simulink model "FOC_core"  (R2025b)
settings: Solver=FixedStepAuto  StartTime=0.0  StopTime=Tstop  FixedStep=p.FastTs  RelTol=1e-3
undefined symbols (not defined in the file): angleDeg, c, Inverter, Motor, p, torqueNm
libraries: fl_lib x4, nesl_utility x3, simulink x2, ee_lib x1
Description:
  | Release 3.0.2
settings Model: Creator=dehc5899  LastModifiedBy=dehc5899
settings SolverCC: AutoInsertRateTranBlk=on
settings DebuggingCC: UnderspecifiedInitializationDetection=Classic

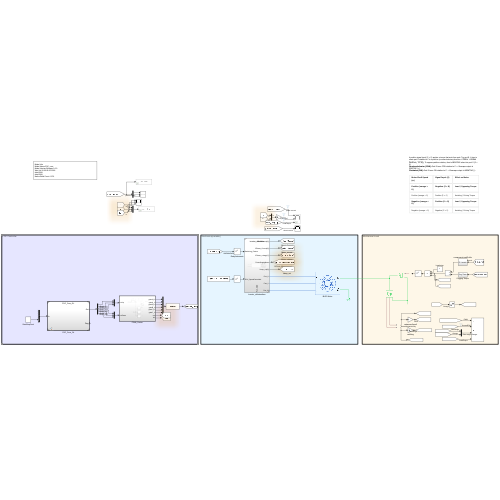
[thumbnail: Simulink's stored preview of the top-level diagram]
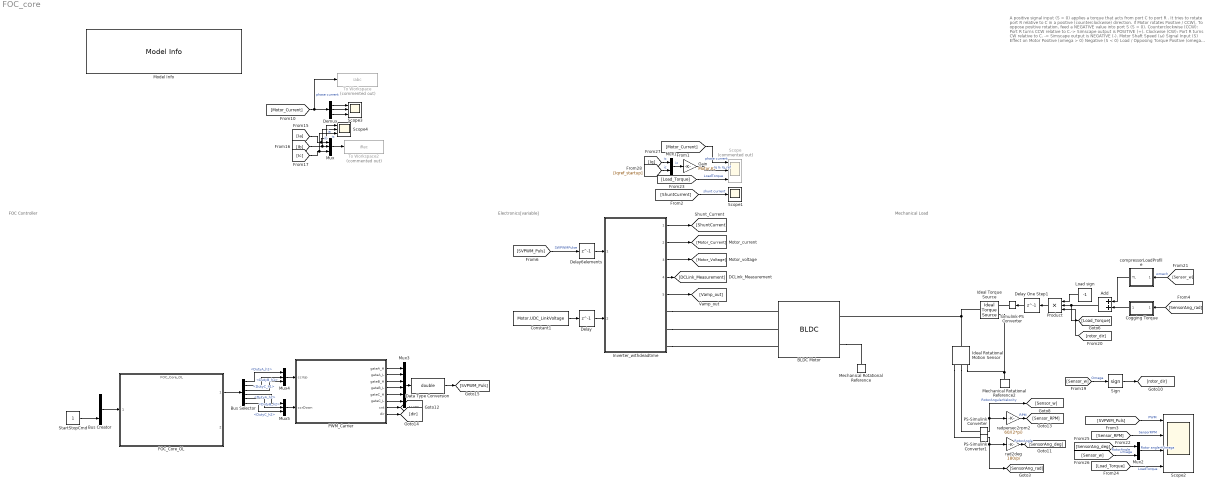
== system FOC_core ==
  note: FOC Controller
  note: A positive signal input (S > 0) applies a torque that acts from port C to port R . It tries to rotate port R relative to C in a positive (counterclockwise) direction. if Motor rotates Positive / CCW), To oppose positive rotation, feed a NEGATIVE value into port S (S < 0).
      | Counterclockwise (CCW): Port R turns CCW relative to C.-> Simscape output is POSITIVE (+).
      | Clockwise (CW): Port R turns CW relative to C. -> Simscape output is NEGATIVE (-).
      |
      | Motor Shaft Speed (ω)
      | Signal Input (S)
      | Effect on Motor
      |
      | Positive (omega > 0)
      | Negative (S < 0)
      | Load / Opposing Torque
      |
      | Positive (omega > 0)
      | Positive (S > 0)
      | Assisting / Driving Torque
      |
      | Negative (omega < 0)
      | Positive (S > 0)
      | Load / Opposing Torque
      |
      | Negative (omega < 0)
      | Negative (S < 0)
      | Assisting / Driving Torque
  note: Electronics[variable]
  note: Mechanical Load
  Add : Sum
  BLDC Motor : ee_lib/Electromechanical/Permanent Magnet/BLDC  port_option=ee.enum.threePhasePort.expanded  rotor_param=ee.enum.pmsm.backemf.tabulatedbackemf  pm_flux_linkage=0.03 Wb  theta_constant=pi / 12 rad  emf_max=9.6 V  w_meas=Motor.bemfMeasSpeed rpm  DphiDtheta_tab=[0, -.1528, -.1528, .1528, .1528, 0] Wb/rad  back_emf_tab=BEMF_shape V  rotor_angle_tab=theta_mech deg  nPolePairs=Motor.PP_NumberOfPolePairs  axes_param=ee.enum.rotorangle.daxis  winding_type=ee.enum.electromech.statorconfiguration.wye  stator_param=ee.enum.statorparam.LsLmMs  machine_param=ee.enum.dqparameterization.constant  Ld=0.00022 H  Lq=0.00022 H  idVec=[-200, 0, 200] A  iqVec=[-200, 0, 200] A  LdMatrix=0.00022 * ones(3, 3) H  LqMatrix=0.00022 * ones(3, 3) H  L0=0.00016 H  Ls=Motor.Ls H  Lm=Motor.Lm H  Ms=Motor.Ms H  Rs=Motor.R_StatorResistance Ohm  zero_sequence=ee.enum.park.zerosequence.exclude  loss_param=ee.enum.ironloss.empirical  losses_oc=[0, 0, 0] W  losses_sc=[0, 0, 0] W  f_losses=60 Hz  Isc_losses=95 A  J=Motor.J_Inertia kg*m^2  lam=Motor.F_FrictionCoeff N*m*s/rad  i_d_specify=off  i_d_priority=None  i_d=0 A  i_d_nominal_specify=off  i_d_nominal_value=1  i_d_nominal_unit=A  i_q_specify=off  i_q_priority=None  i_q=0 A  i_q_nominal_specify=off  i_q_nominal_value=1  i_q_nominal_unit=A  torque_specify=off  torque_priority=None  torque=0 N*m  torque_nominal_specify=off  torque_nominal_value=1  torque_nominal_unit=N*m  angular_velocity_specify=on  angular_velocity_priority=Low  angular_velocity=Motor.wm0_InitialRotorSpeed rpm  angular_velocity_nominal_specify=off  angular_velocity_nominal_value=Motor.nNom_NominalSpeedrpm  angular_velocity_nominal_unit=rpm  angular_position_specify=on  angular_position_priority=Low  angular_position=Motor.thm0_InitialRotorAngle rad  angular_position_nominal_specify=off  angular_position_nominal_value=Motor.thm0_InitialRotorAngle  angular_position_nominal_unit=deg  alpha=3.93e-3 1/K  alpha_flux=-0.001 1/K  Tmeas=298.15 K  stator_thermal_mass=100 J/K  rotor_thermal_mass=200 J/K  Rm_percent_rotor=90  Rd_percent_rotor=30  temperatureA_specify=off  temperatureA_priority=High  temperatureA=25 degC  temperatureA_nominal_specify=off  temperatureA_nominal_value=1  temperatureA_nominal_unit=degC  temperatureB_specify=off  temperatureB_priority=High  temperatureB=25 degC  temperatureB_nominal_specify=off  temperatureB_nominal_value=1  temperatureB_nominal_unit=degC  temperatureC_specify=off  temperatureC_priority=High  temperatureC=25 degC  temperatureC_nominal_specify=off  temperatureC_nominal_value=1  temperatureC_nominal_unit=degC  temperatureR_specify=off  temperatureR_priority=High  temperatureR=25 degC  temperatureR_nominal_specify=off  temperatureR_nominal_value=1  temperatureR_nominal_unit=degC
      settings: InternalSimscapePortConfiguration="{\"Bottom\":[],\"Left\":[{\"id\":\"a\",\"label\":\"a\",\"type\":\"foundation.electrical.electrical\"},{\"id\":\"b\",\"label\":\"b\",\"type\":\"foundation.electrical.electrical\"},{\"id\":\"c\",\"label\":\"c\",\"type\":\"foundation.electrical.electrical\"}],\"Right\":[{\"id\":\"R\",\"label\":\"R\",\"type\":\"foundation.mechanical.rotational.rotational\"},{\"id\":\"C\",\"label\":\"C\",\"type\":\"foundation.mechanical.rotational.rotational\"}],\"Top\":[]}"
  Bus Creator : BusCreator  Inputs=7  OutDataTypeStr=Bus: FOC_Inputs_t
  Bus Selector : BusSelector  OutputSignals=DutyA_h1,DutyB_h1,DutyC_h1,DutyA_h2,DutyB_h2,DutyC_h2
  Cogging Torque : Subsystem
      settings: PortSchema="{\"entries\":[{\"content\":{\"sides\":[{\"content\":{\"connectorIds\":[\"Out1\"]},\"type\":\"ConnectorPlacement.EquallySpacedRectSide\",\"uuid\":\"e72dd149-be6c-473d-b9a6-ab382dc36dd8\"},{\"content\":{\"connectorIds\":[\"In1\"],\"side\":\"RIGHT\"},\"type\":\"ConnectorPlacement.EquallySpacedRectSide\",\"uuid\":\"d6dbddf8-c929-46f7-8e18-d8605da261d8\"},{\"content\":{\"side\":\"TOP\"},\"type\":\"ConnectorPlacement.EquallySpacedRectSide\",\"uuid\":\"d97b9a66-7b14-44a9-8763-71570facd52d\"},{\"content\":{\"side\":\"BOTTOM\"},\"type\":\"ConnectorPlacement.EquallySpacedRectSide\",\"uuid\":\"30e90f76-fd4e-40c6-9e4e-ba219d693512\"}]},\"type\":\"ConnectorPlacement.EquallySpacedConnector\",\"uuid\":\"ce9d67e2-aed0-4e64-a6bd-15c2f7731a50\"}],\"packageUris\":[\"http://schema.mathworks.com/mf0/Connector/R2020b\"],\"version\":\"1.0\"}"
  Constant1 : Constant  Value=Motor.UDC_LinkVoltage
  Data Type Conversion : DataTypeConversion  OutDataTypeStr=double  SaturateOnIntegerOverflow=off  RndMeth=Floor
  Delay : Delay  DelayLength=1  InitialCondition=Inverter.UDC_LinkVoltage_Max  InputProcessing=Columns as channels (frame based)
  Delay One Step1 : Delay  DelayLength=1
  Delay6elements : Delay  DelayLength=1  InitialCondition=[0 0 0 0 0 0]
  Demux : Demux  Outputs=3
  FOC_Core_OL : ModelReference  ModelNameDialog=FOC_Core_OL  SimulationMode=Normal  ModelReferenceVersion=1.291
  Gain : Gain  Gain=Motor.Kt
  Ideal Rotational Motion Sensor : fl_lib/Mechanical/Mechanical Sensors/Ideal Rotational Motion Sensor  reference=foundation.enum.MeasurementReference.difference  acceleration_port=false  velocity_port=true  position_port=true  wrap_angle=true  offset=Motor.thm0_InitialRotorAngle rad
  Ideal Torque Source : fl_lib/Mechanical/Mechanical Sources/Ideal Torque Source
  Inverter_withdeadtime : Subsystem  ReferencedSubsystem=inverter_withdtime
      settings: PortSchema="{\"entries\":[{\"content\":{\"sides\":[{\"content\":{\"connectorIds\":[\"In1\",\"In2\"]},\"type\":\"ConnectorPlacement.EquallySpacedRectSide\",\"uuid\":\"c4e4a499-a73b-47b6-b9d4-05a0b5c00da1\"},{\"content\":{\"connectorIds\":[\"Out1\",\"Out2\",\"Out3\",\"Out4\",\"Out5\",\"RConn1\",\"RConn2\",\"RConn3\"],\"side\":\"RIGHT\"},\"type\":\"ConnectorPlacement.EquallySpacedRectSide\",\"uuid\":\"f55443ed-1206-46a2-9a95-70ed1e950cf9\"},{\"content\":{\"side\":\"TOP\"},\"type\":\"ConnectorPlacement.EquallySpacedRectSide\",\"uuid\":\"cf76199e-050b-45cf-ab73-853bf2c84fa8\"},{\"content\":{\"connectorIds\":[\"RConn4\"],\"side\":\"BOTTOM\"},\"type\":\"ConnectorPlacement.EquallySpacedRectSide\",\"uuid\":\"91869a37-cdc1-4525-aadb-c80a51613b54\"}]},\"type\":\"ConnectorPlacement.EquallySpacedConnector\",\"uuid\":\"fb7c01bd-e96a-47ac-9a1b-b2a6f4f5bd80\"}],\"packageUris\":[\"http://schema.mathworks.com/mf0/Connector/R2020b\"],\"version\":\"1.0\"}"
  Load sign : Constant  Value=-1
  Mechanical Rotational Reference : fl_lib/Mechanical/Rotational Elements/Mechanical Rotational Reference
  Mechanical Rotational Reference2 : fl_lib/Mechanical/Rotational Elements/Mechanical Rotational Reference
  Model Info : simulink/Model-Wide Utilities/Model Info  Frame=on  DisplayStringWithTags=|  HorizontalTextAlignment=Left  LeftAlignmentValue=0.02
      | Model Info
      | Model Name:%<ModelName>
      | Model Version:%<Description>
      | %<Created>
      | %<Creator>
      | %<LastModifiedBy>
      | Native Build Count:%<ModelVersion>
  Mux : Mux  Inputs=3
  Mux1 : Mux  Inputs=2
  Mux2 : Mux  Inputs=2
  Mux3 : Mux  Inputs=6
  Mux4 : Mux  Inputs=3
  Mux5 : Mux  Inputs=3
  PS-Simulink Converter : nesl_utility/PS-Simulink Converter  PhysicalDomain=network_engine_domain  SubClassName=ps_output  LeftPortType=input  RightPortType=output  PseudoPeriodic=off  Frequencies=[]  VectorFormat=inherit  Unit=inherit  AffineConversion=off
  PS-Simulink Converter1 : nesl_utility/PS-Simulink Converter  PhysicalDomain=network_engine_domain  SubClassName=ps_output  LeftPortType=input  RightPortType=output  PseudoPeriodic=off  Frequencies=[]  VectorFormat=inherit  Unit=inherit  AffineConversion=off
  PWM_Carrier : Subsystem  TreatAsAtomicUnit=on  SystemSampleTime=p.FastTs
  Product : Product  Inputs=3
  Scope : Scope  Commented=on  NumInputPorts=3
      settings: ActiveDisplayYMinimum=-25.470769165207408  ActiveDisplayYMaximum=27.204092861454868  DataLoggingVariableName=ScopeData4
  Scope1 : Scope
      settings: ActiveDisplayYMinimum=-6.3618713706725121  ActiveDisplayYMaximum=11.690256831370988  DataLoggingVariableName=ScopeData9
  Scope2 : Scope  NumInputPorts=4
      settings: ActiveDisplayYMinimum=-0.12499999999999997  ActiveDisplayYMaximum=1.125  DataLoggingVariableName=ScopeData5
  Scope3 : Scope  NumInputPorts=3
      settings: ActiveDisplayYMinimum=-12.058935324686422  ActiveDisplayYMaximum=12.950717402584473  DataLoggingVariableName=ScopeData23
  Scope4 : Scope  NumInputPorts=3
      settings: ActiveDisplayYMinimum=-2.083290326404279  ActiveDisplayYMaximum=1.1649120394540577  DataLoggingVariableName=ScopeData17
  Sign : Signum
  Simulink-PS Converter : nesl_utility/Simulink-PS Converter  PhysicalDomain=network_engine_domain  SubClassName=ps_input  LeftPortType=input  RightPortType=output  PseudoPeriodic=off  Frequencies=[]  NoiseDistribution=none  NoiseParameters=[]  Unit=1  AffineConversion=off  FilteringAndDerivatives=provide  SimscapeFilterOrder=1  InputFilterTimeConstant=0.001  UdotUserProvided=0
  StartStopCmd : Constant  OutDataTypeStr=uint8
  To Workspace : ToWorkspace  Commented=on  VariableName=iabc  SaveFormat=Timeseries  SampleTime=-1
  To Workspace2 : ToWorkspace  Commented=on  VariableName=iRec  SaveFormat=Timeseries  SampleTime=-1
  compressorLoadProfile : Subsystem
  rad2deg : Gain  Gain=180/pi
  radpersec2rpm2 : Gain  Gain=60/(2*pi)
  wires:
  Inverter_withdeadtime/4 -> [DCLink_Measurement]
  [SVPWM_Puls] -> Delay6elements/1  "SWPWMPulse"
  Inverter_withdeadtime/3 -> [Motor_Voltage]
  Inverter_withdeadtime/2 -> [Motor_Current]
  Inverter_withdeadtime/1 -> [ShuntCurrent]
  Delay/1 -> Inverter_withdeadtime/2
  Constant1/1 -> Delay/1
  Delay6elements/1 -> Inverter_withdeadtime/1
  [SensorAng_rad] -> Cogging Torque/1(Theta)
  PS-Simulink Converter/1 -> radpersec2rpm2/1, [Sensor_w]  "RotorAngularVelocity"
  rad2deg/1 -> [SensorAng_deg]  "RotorAngle"
  [Load_Torque] -> Scope2/4  "LoadTorque"
  PS-Simulink Converter1/1 -> [SensorAng_rad], rad2deg/1
  [Sensor_w] -> Mux2/2  "Omega"
  Cogging Torque/1(Tcog) -> Add/2
  Add/1 -> Product/2, [Load_Torque]
  [SensorAng_deg] -> Mux2/1  "RotorAngle"
  [SVPWM_Puls] -> Scope2/1  "PWM"
  radpersec2rpm2/1 -> [Sensor_RPM]  "RPM"
  Mux2/1 -> Scope2/3  "Rotor angle+Omega"
  [Sensor_RPM] -> Scope2/2  "SensorRPM"
  [Motor_Current] -> Scope/1  "phase current"
  [ShuntCurrent] -> Scope1/1  "shunt current"
  Inverter_withdeadtime/5 -> [Vamp_out]
  [Ib] -> Scope4/2, Mux/2  "ib"
  [Ia] -> Scope4/1, Mux/1  "ia"
  [Ic] -> Scope4/3, Mux/3  "ic"
  [Motor_Current] -> To Workspace/1, Demux/1  "phase current"
  Demux/1 -> Scope3/1
  Demux/2 -> Scope3/2
  Demux/3 -> Scope3/3
  Mux/1 -> To Workspace2/1
  Product/1 -> Delay One Step1/1
  [Sensor_w] -> Sign/1  "Omega"
  Sign/1 -> [rotor_dir]
  Load sign/1 -> Product/1
  [rotor_dir] -> Product/3
  Delay One Step1/1 -> Simulink-PS Converter/1
  [Sensor_w] -> compressorLoadProfile/1(wmech)  "wmech"
  compressorLoadProfile/1(TL) -> Add/1
  [Load_Torque] -> Scope/3  "LoadTorque"
  Mux1/1 -> Gain/1  "ic"
  Gain/1 -> Scope/2  "Iq & Iq_ref"
  [Iq] -> Mux1/1  "ic"
  [Iqref_startup] -> Mux1/2  "ic"
  PWM_Carrier/2(gateA_L) -> Mux3/2
  PWM_Carrier/5(gateC_H) -> Mux3/5
  PWM_Carrier/1(gateA_H) -> Mux3/1
  PWM_Carrier/7(cnt) -> [cnt]
  PWM_Carrier/6(gateC_L) -> Mux3/6
  PWM_Carrier/3(gateB_H) -> Mux3/3
  PWM_Carrier/4(gateB_L) -> Mux3/4
  Data Type Conversion/1 -> [SVPWM_Puls]
  PWM_Carrier/8(dir) -> [dir]
  Mux3/1 -> Data Type Conversion/1
  FOC_Core_OL/1 -> Bus Selector/1
  Bus Creator/1 -> FOC_Core_OL/1
  Mux4/1 -> PWM_Carrier/1(ccrUp)
  Bus Selector/1 -> Mux4/1  "<DutyA_h1>"
  Bus Selector/2 -> Mux4/2  "<DutyB_h1>"
  Bus Selector/3 -> Mux4/3  "<DutyC_h1>"
  Bus Selector/4 -> Mux5/1  "<DutyA_h2>"
  Bus Selector/5 -> Mux5/2  "<DutyB_h2>"
  Bus Selector/6 -> Mux5/3  "<DutyC_h2>"
  Mux5/1 -> PWM_Carrier/2(ccrDown)
  StartStopCmd/1 -> Bus Creator/6
  connections:
  BLDC Motor/RConn2 -- Mechanical Rotational Reference/LConn1
  Inverter_withdeadtime/RConn1 -- BLDC Motor/LConn1
  Inverter_withdeadtime/RConn2 -- BLDC Motor/LConn2
  Inverter_withdeadtime/RConn3 -- BLDC Motor/LConn3
  Mechanical Rotational Reference2/LConn1 -- Ideal Rotational Motion Sensor/RConn1 -- Ideal Torque Source/RConn2
  Ideal Torque Source/LConn1 -- Ideal Rotational Motion Sensor/LConn1 -- BLDC Motor/RConn1
  Ideal Rotational Motion Sensor/RConn3 -- PS-Simulink Converter1/LConn1
  Ideal Rotational Motion Sensor/RConn2 -- PS-Simulink Converter/LConn1
  Simulink-PS Converter/RConn1 -- Ideal Torque Source/RConn1

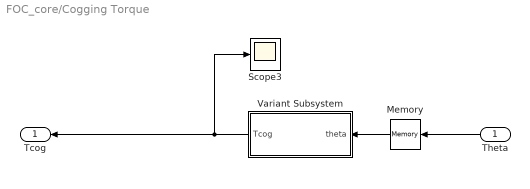
== system FOC_core/Cogging Torque ==
  Theta : Inport
  Memory : Memory
  Scope3 : Scope
      settings: ActiveDisplayYMinimum=-0.048749999766971877  ActiveDisplayYMaximum=0.048749999963062271  DataLoggingVariableName=ScopeData6
  Variant Subsystem : Subsystem  Variant=on  EmptyChoice=on
  Tcog : Outport
  wires:
  Theta/1 -> Memory/1
  Variant Subsystem/1(Tcog) -> Scope3/1, Tcog/1
  Memory/1 -> Variant Subsystem/1(theta)

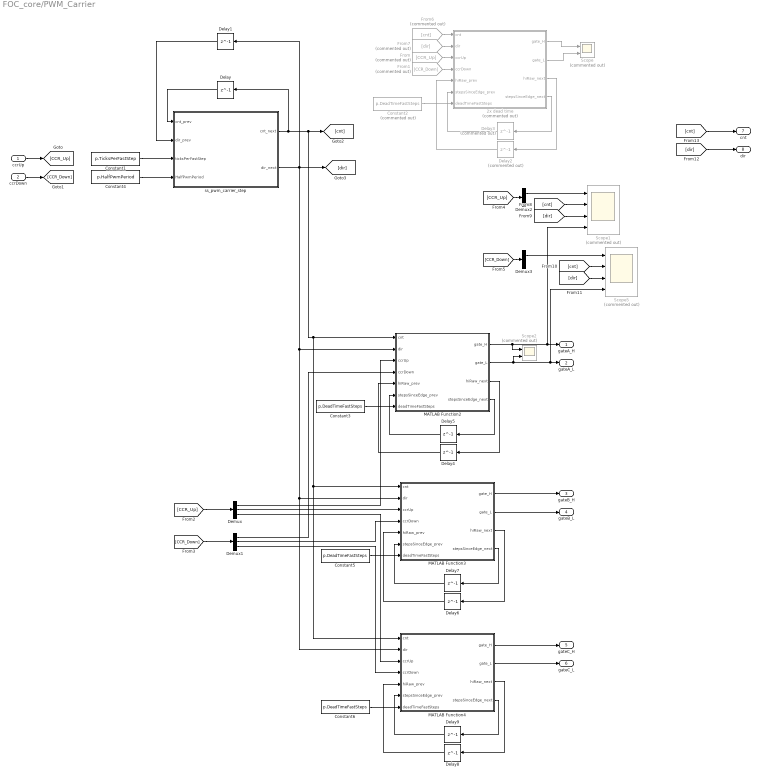
== system FOC_core/PWM_Carrier ==
  ccrUp : Inport
  ccrDown : Inport  Port=2
  2x dead time : MATLAB Function  Commented=on  TreatAsAtomicUnit=on
  Constant1 : Constant  Value=p.TicksPerFastStep
  Constant2 : Constant  Commented=on  Value=p.DeadTimeFastSteps
  Constant3 : Constant  Value=p.DeadTimeFastSteps
  Constant4 : Constant  Value=p.HalfPwmPeriod
  Constant5 : Constant  Value=p.DeadTimeFastSteps
  Constant6 : Constant  Value=p.DeadTimeFastSteps
  Delay{,4..9} (7 alike) : Delay  DelayLength=1  SampleTime=p.FastTs
  Delay1 : Delay  DelayLength=1  InitialCondition=1  SampleTime=p.FastTs
  Delay2 : Delay  Commented=on  DelayLength=1  SampleTime=p.FastTs
  Delay3 : Delay  Commented=on  DelayLength=1  SampleTime=p.FastTs
  Demux{,1..3} (4 alike) : Demux  Outputs=3
  From : From  Commented=on  GotoTag=CCR_Up
  From1 : From  Commented=on  GotoTag=CCR_Down
  From6 : From  Commented=on  GotoTag=cnt
  From7 : From  Commented=on  GotoTag=dir
  MATLAB Function2 : MATLAB Function  TreatAsAtomicUnit=on
  MATLAB Function3 : MATLAB Function  TreatAsAtomicUnit=on
  MATLAB Function4 : MATLAB Function  TreatAsAtomicUnit=on
  Scope : Scope  Commented=on  NumInputPorts=2
      settings: ActiveDisplayYMinimum=-0.12499999999999997  ActiveDisplayYMaximum=1.125  DataLoggingVariableName=ScopeData14
  Scope1 : Scope  Commented=on  NumInputPorts=4
      settings: ActiveDisplayYMinimum=-9127.6330234277448  ActiveDisplayYMaximum=17916.94761530693  DataLoggingVariableName=ScopeData13
  Scope2 : Scope  Commented=on  NumInputPorts=2
      settings: ActiveDisplayYMinimum=-0.12499999999999997  ActiveDisplayYMaximum=1.125  DataLoggingVariableName=ScopeData21
  Scope5 : Scope  Commented=on  NumInputPorts=4
      settings: ActiveDisplayYMinimum=-665.124999999998  ActiveDisplayYMaximum=5976.1249999999827  DataLoggingVariableName=ScopeData18
  ss_pwm_carrier_step : MATLAB Function  TreatAsAtomicUnit=on
  gateA_H : Outport
  gateA_L : Outport  Port=2
  gateB_H : Outport  Port=3
  gateB_L : Outport  Port=4
  gateC_H : Outport  Port=5
  gateC_L : Outport  Port=6
  cnt : Outport  Port=7
  dir : Outport  Port=8
  wires:
  Constant4/1 -> ss_pwm_carrier_step/4(HalfPwmPeriod)
  Constant1/1 -> ss_pwm_carrier_step/3(ticksPerFastStep)
  Delay/1 -> ss_pwm_carrier_step/1(cnt_prev)
  Delay1/1 -> ss_pwm_carrier_step/2(dir_prev)
  2x dead time/3(hiRaw_next) -> Delay2/1
  Delay2/1 -> 2x dead time/5(hiRaw_prev)
  2x dead time/4(stepsSinceEdge_next) -> Delay3/1
  Delay3/1 -> 2x dead time/6(stepsSinceEdge_prev)
  Constant2/1 -> 2x dead time/7(deadTimeFastSteps)
  2x dead time/1(gate_H) -> Scope/1
  2x dead time/2(gate_L) -> Scope/2
  ccrUp/1 -> [CCR_Up]
  ccrDown/1 -> [CCR_Down]
  From/1 -> 2x dead time/3(ccrUp)
  From1/1 -> 2x dead time/4(ccrDown)
  [CCR_Up] -> Demux/1
  [CCR_Down] -> Demux1/1
  Demux1/1 -> MATLAB Function2/4(ccrDown)
  Demux/1 -> MATLAB Function2/3(ccrUp)
  MATLAB Function2/2(gate_L) -> Scope2/2, Scope5/4, gateA_L/1
  MATLAB Function2/1(gate_H) -> Scope2/1, gateA_H/1, Scope1/4
  Constant3/1 -> MATLAB Function2/7(deadTimeFastSteps)
  Delay5/1 -> MATLAB Function2/6(stepsSinceEdge_prev)
  MATLAB Function2/4(stepsSinceEdge_next) -> Delay5/1
  Delay4/1 -> MATLAB Function2/5(hiRaw_prev)
  MATLAB Function2/3(hiRaw_next) -> Delay4/1
  MATLAB Function3/3(hiRaw_next) -> Delay6/1
  Delay6/1 -> MATLAB Function3/5(hiRaw_prev)
  MATLAB Function3/4(stepsSinceEdge_next) -> Delay7/1
  Delay7/1 -> MATLAB Function3/6(stepsSinceEdge_prev)
  Constant5/1 -> MATLAB Function3/7(deadTimeFastSteps)
  MATLAB Function3/1(gate_H) -> gateB_H/1
  MATLAB Function3/2(gate_L) -> gateB_L/1
  Demux/2 -> MATLAB Function3/3(ccrUp)
  Demux1/2 -> MATLAB Function3/4(ccrDown)
  Demux1/3 -> MATLAB Function4/4(ccrDown)
  Demux/3 -> MATLAB Function4/3(ccrUp)
  MATLAB Function4/2(gate_L) -> gateC_L/1
  MATLAB Function4/1(gate_H) -> gateC_H/1
  Constant6/1 -> MATLAB Function4/7(deadTimeFastSteps)
  Delay9/1 -> MATLAB Function4/6(stepsSinceEdge_prev)
  MATLAB Function4/4(stepsSinceEdge_next) -> Delay9/1
  Delay8/1 -> MATLAB Function4/5(hiRaw_prev)
  MATLAB Function4/3(hiRaw_next) -> Delay8/1
  ss_pwm_carrier_step/2(dir_next) -> [dir], Delay1/1, MATLAB Function2/2(dir), MATLAB Function3/2(dir), MATLAB Function4/2(dir)
  ss_pwm_carrier_step/1(cnt_next) -> MATLAB Function4/1(cnt), MATLAB Function3/1(cnt), MATLAB Function2/1(cnt), [cnt], Delay/1
  [CCR_Up] -> Demux2/1
  [CCR_Down] -> Demux3/1
  Demux2/1 -> Scope1/1
  Demux3/1 -> Scope5/1
  From6/1 -> 2x dead time/1(cnt)
  From7/1 -> 2x dead time/2(dir)
  [cnt] -> Scope1/2
  [dir] -> Scope1/3
  [dir] -> Scope5/3
  [cnt] -> Scope5/2
  [cnt] -> cnt/1
  [dir] -> dir/1

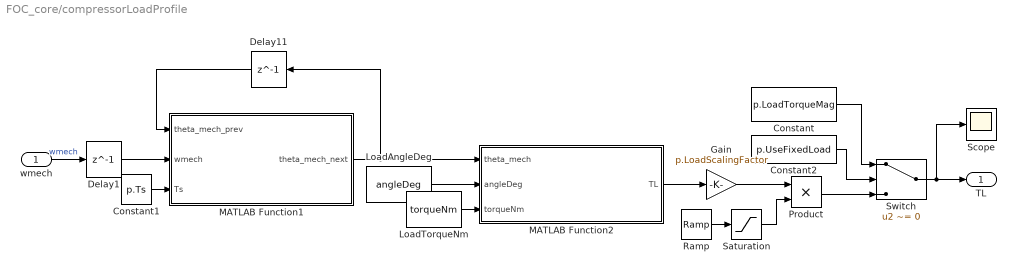
== system FOC_core/compressorLoadProfile ==
  wmech : Inport
  Constant : Constant  Value=p.LoadTorqueMag
  Constant1 : Constant  Value=p.Ts
  Constant2 : Constant  Value=p.UseFixedLoad
  Delay1 : Delay  DelayLength=1  SampleTime=p.Ts
  Delay11 : Delay  DelayLength=1  SampleTime=p.Ts
  Gain : Gain  Gain=p.LoadScalingFactor
  LoadAngleDeg : Constant  Value=angleDeg
  LoadTorqueNm : Constant  Value=torqueNm
  MATLAB Function1 : MATLAB Function  TreatAsAtomicUnit=on
  MATLAB Function2 : MATLAB Function  TreatAsAtomicUnit=on
  Product : Product
  Ramp : simulink/Sources/Ramp  slope=p.loadRampSlope  start=p.Startup_T(1)  InitialOutput=0
  Saturation : Saturate  UpperLimit=1  LowerLimit=0
  Scope : Scope
      settings: ActiveDisplayYMinimum=-1  ActiveDisplayYMaximum=1  DataLoggingVariableName=ScopeData41
  Switch : Switch  Criteria=u2 ~= 0  SaturateOnIntegerOverflow=off  InputSameDT=off
  TL : Outport
  wires:
  Constant1/1 -> MATLAB Function1/3(Ts)
  LoadAngleDeg/1 -> MATLAB Function2/2(angleDeg)
  LoadTorqueNm/1 -> MATLAB Function2/3(torqueNm)
  wmech/1 -> Delay1/1  "wmech"
  MATLAB Function1/1(theta_mech_next) -> MATLAB Function2/1(theta_mech), Delay11/1
  Delay11/1 -> MATLAB Function1/1(theta_mech_prev)
  MATLAB Function2/1(TL) -> Gain/1
  Delay1/1 -> MATLAB Function1/2(wmech)
  Ramp/1 -> Saturation/1
  Saturation/1 -> Product/2
  Constant2/1 -> Switch/2
  Product/1 -> Switch/3
  Constant/1 -> Switch/1
  Switch/1 -> Scope/1, TL/1
  Gain/1 -> Product/1

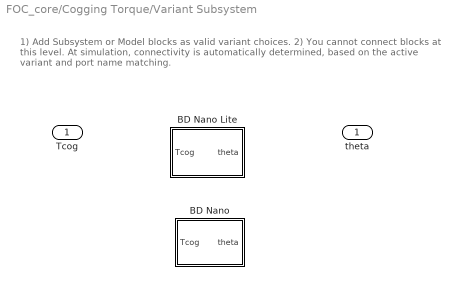
== system FOC_core/Cogging Torque/Variant Subsystem ==
  note: 1) Add Subsystem or Model blocks as valid variant choices.
      | 2) You cannot connect blocks at this level. At simulation, connectivity is automatically
      | determined, based on the active variant and port name matching.
  theta : Inport
  BD Nano : Subsystem  VariantControl=Option.Product==1
  BD Nano Lite : Subsystem  VariantControl=Option.Product==4
  Tcog : Outport

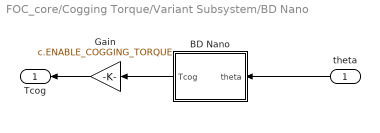
== system FOC_core/Cogging Torque/Variant Subsystem/BD Nano ==
  theta : Inport
  BD Nano : MATLAB Function  TreatAsAtomicUnit=on  VariantControl=Option.Product==1
  Gain : Gain  Gain=c.ENABLE_COGGING_TORQUE
  Tcog : Outport
  wires:
  BD Nano/1(Tcog) -> Gain/1
  theta/1 -> BD Nano/1(theta)
  Gain/1 -> Tcog/1

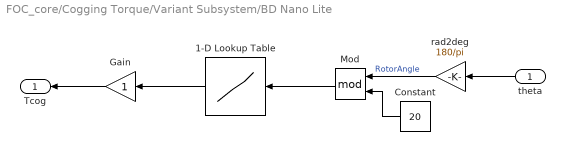
== system FOC_core/Cogging Torque/Variant Subsystem/BD Nano Lite ==
  theta : Inport
  1-D Lookup Table : Lookup_n-D  NumberOfTableDimensions=1  BreakpointsForDimension1=|  BreakpointsForDimension1FirstPoint=0  BreakpointsForDimension1Spacing=0.5  Table=|  InterpMethod=Cubic spline  ExtrapMethod=Cubic spline  InternalRulePriority=Speed  RndMeth=Simplest
      BreakpointsForDimension1=|
      | [0.0
      | 0.5
      | 1.0
      | 1.5
      | 2.0
      | 2.5
      | 3.0
      | 3.5
      | 4.0
      | 4.5
      | 5.0
      | 5.5
      | 6.0
      | 6.5
      | 7.0
      | 7.5
      | 8.0
      | 8.5
      | 9.0
      | 9.5
      | 10.0
      | 10.5
      | 11.0
      | 11.5
      | 12.0
      | 12.5
      | 13.0
      | 13.5
      | 14.0
      | 14.5
      | 15.0
      | 15.5
      | 16.0
      | 16.5
      | 17.0
      | 17.5
      | 18.0
      | 18.5
      | 19.0
      | 19.5
      | 20.0]
      Table=|
      | [0.001
      | 0.002
      | 0.003
      | 0.004
      | 0.005
      | 0.007
      | 0.009
      | 0.011
      | 0.013
      | 0.015
      | 0.017
      | 0.018
      | 0.019
      | 0.018
      | 0.016
      | 0.013
      | 0.010
      | 0.007
      | 0.005
      | 0.003
      | 0.002
      | 0.001
      | 0.000
      | -0.002
      | -0.004
      | -0.007
      | -0.010
      | -0.014
      | -0.017
      | -0.019
      | -0.020
      | -0.019
      | -0.018
      | -0.016
      | -0.014
      | -0.012
      | -0.010
      | -0.008
      | -0.006
      | -0.004
      | -0.001]
  Constant : Constant  Value=20
  Gain : Gain
  Mod : Math  Operator=mod
  rad2deg : Gain  Gain=180/pi
  Tcog : Outport
  wires:
  theta/1 -> rad2deg/1
  1-D Lookup Table/1 -> Gain/1
  Mod/1 -> 1-D Lookup Table/1
  rad2deg/1 -> Mod/1  "RotorAngle"
  Constant/1 -> Mod/2
  Gain/1 -> Tcog/1

== matlab function FOC_core/compressorLoadProfile/MATLAB Function2 ==
  data: theta_mech input; TL output; angleDeg input; torqueNm input
function TL = ss_load_torque_lookup(theta_mech, angleDeg, torqueNm)
%SS_LOAD_TORQUE_LOOKUP Interpolates the measured load-torque-vs-crank-
% angle table (ss_load_torque_data.m) at the current mechanical angle.
%
% theta_mech : mechanical crank angle, radians, wrapped [0, 2*pi) - feed
%              the DELAYED ss_mech_angle_step.m state (theta_mech_prev),
%              NOT its just-computed theta_mech_next: this value has to
%              be available to compute THIS period's TL feeding
%              ss_mechanical_model.m, which is what produces the speed
%              theta_mech_next is integrated from - using the delayed
%              state avoids a zero-delay algebraic loop, same principle
%              as everywhere else in this build.
% angleDeg, torqueNm : ss_load_torque_data.m output - feed via two
%              Constant blocks (e.g. LoadAngleDeg, LoadTorqueNm), NOT
%              recomputed every step
%
% TL : load torque, Nm, at this instant - feed into
%      ss_mechanical_model.m's TL input (replacing the constant 0.11/0)

theta_deg = mod(theta_mech * 180/pi, 360);
TL = interp1(angleDeg, torqueNm, theta_deg, 'linear');

end

== matlab function FOC_core/PWM_Carrier/2x dead time ==
  data: cnt input; gate_H output; dir input; ccrUp input; ccrDown input; hiRaw_prev input double; stepsSinceEdge_prev input double; deadTimeFastSteps input; gate_L output; hiRaw_next output; stepsSinceEdge_next output
function [gate_H, gate_L, hiRaw_next, stepsSinceEdge_next] = ss_pwm_gate_step( ...
    cnt, dir, ccrUp, ccrDown, hiRaw_prev, stepsSinceEdge_prev, deadTimeFastSteps)
%SS_PWM_GATE_STEP One fast-rate (p.FastTs) step of a single phase's
% high/low-side switch state, matching STM32 timer PWM mode 1 (active
% while counter < compare value, regardless of counting direction) with
% dead-time inserted around every transition.
%
% Call this once per phase (A/B/C) each fast step - each phase has its
% own hiRaw_prev/stepsSinceEdge_prev state, fed back through Unit Delay
% (Z^-1) blocks AT THE FAST RATE, initial condition hiRaw=false,
% stepsSinceEdge=deadTimeFastSteps (so the very first step isn't wrongly
% held in a dead zone).
%
% This is a genuinely stateful, one-fast-step-at-a-time replacement for
% ss_pwm_waveform.m's batch/offline NxN dead-time trick - simpler and
% more natural now that this runs as part of the live simulation instead
% of a one-shot reconstruction: "how many fast steps since the last
% transition" is just a counter, no need to find edges after the fact.
%
% cnt, dir            : ss_pwm_carrier_step.m output, this fast step
% ccrUp, ccrDown       : this phase's compare value for the up-count/
%                        down-count half (ss_calc_duty_and_samplepoints.m's
%                        DmaBuffCCR_up(k)/DmaBuffCCR_down(k), HELD constant
%                        across the whole PWM period via a Rate Transition
%                        block from the slow p.Ts domain)
% hiRaw_prev           : previous fast step's un-gated compare result
%                        (before dead-time), for edge detection
% stepsSinceEdge_prev  : fast steps elapsed since the last transition
% deadTimeFastSteps    : p.DeadTimeFastSteps
%
% gate_H, gate_L       : dead-time-gated high/low-side switch state
% hiRaw_next, stepsSinceEdge_next : feed back to next fast step

if dir > 0
    hiRaw_next = double(cnt < ccrUp);
else
    hiRaw_next = double(cnt < ccrDown);
end

if hiRaw_next ~= hiRaw_prev
    stepsSinceEdge_next = double(0);
else
    stepsSinceEdge_next = double(stepsSinceEdge_prev + 1);
end

inDeadZone = stepsSinceEdge_next <= deadTimeFastSteps;

gate_H = double(hiRaw_next & ~inDeadZone);
gate_L = double(~hiRaw_next & ~inDeadZone);

end

== matlab function FOC_core/PWM_Carrier/MATLAB Function2 ==
  data: cnt input; gate_H output double; dir input; ccrUp input; ccrDown input; hiRaw_prev input double; stepsSinceEdge_prev input double; deadTimeFastSteps input; gate_L output double; hiRaw_next output; stepsSinceEdge_next output
function [gate_H, gate_L, hiRaw_next, stepsSinceEdge_next] = ss_pwm_gate_step( ...
    cnt, dir, ccrUp, ccrDown, hiRaw_prev, stepsSinceEdge_prev, deadTimeFastSteps)
%SS_PWM_GATE_STEP One fast-rate (p.FastTs) step of a single phase's
% high/low-side switch state, matching STM32 timer PWM mode 1 (active
% while counter < compare value, regardless of counting direction) with
% dead-time inserted around every transition.
%
% Call this once per phase (A/B/C) each fast step - each phase has its
% own hiRaw_prev/stepsSinceEdge_prev state, fed back through Unit Delay
% (Z^-1) blocks AT THE FAST RATE, initial condition hiRaw=false,
% stepsSinceEdge=deadTimeFastSteps (so the very first step isn't wrongly
% held in a dead zone).
%
% This is a genuinely stateful, one-fast-step-at-a-time replacement for
% ss_pwm_waveform.m's batch/offline NxN dead-time trick - simpler and
% more natural now that this runs as part of the live simulation instead
% of a one-shot reconstruction: "how many fast steps since the last
% transition" is just a counter, no need to find edges after the fact.
%
% cnt, dir            : ss_pwm_carrier_step.m output, this fast step
% ccrUp, ccrDown       : this phase's compare value for the up-count/
%                        down-count half (ss_calc_duty_and_samplepoints.m's
%                        DmaBuffCCR_up(k)/DmaBuffCCR_down(k), HELD constant
%                        across the whole PWM period via a Rate Transition
%                        block from the slow p.Ts domain)
% hiRaw_prev           : previous fast step's un-gated compare result
%                        (before dead-time), for edge detection
% stepsSinceEdge_prev  : fast steps elapsed since the last transition
% deadTimeFastSteps    : p.DeadTimeFastSteps
%
% gate_H, gate_L       : dead-time-gated high/low-side switch state
% hiRaw_next, stepsSinceEdge_next : feed back to next fast step

if dir > 0
    hiRaw_next = double(cnt < ccrUp);
else
    hiRaw_next = double(cnt < ccrDown);
end

if hiRaw_next ~= hiRaw_prev
    stepsSinceEdge_next = double(0);
else
    stepsSinceEdge_next = double(stepsSinceEdge_prev + 1);
end

inDeadZone = stepsSinceEdge_next < deadTimeFastSteps;

gate_H = double(hiRaw_next & ~inDeadZone);
gate_L = double(~hiRaw_next & ~inDeadZone);

end

== matlab function FOC_core/Cogging Torque/Variant Subsystem/BD Nano/BD Nano ==
  data: theta input size=1; Tcog output size=1
function Tcog = fcn(theta)

Tcog = 0.039*sin(18*theta);

== matlab function FOC_core/PWM_Carrier/MATLAB Function3 ==
  data: cnt input; gate_H output double; dir input; ccrUp input; ccrDown input; hiRaw_prev input double; stepsSinceEdge_prev input double; deadTimeFastSteps input; gate_L output double; hiRaw_next output; stepsSinceEdge_next output
function [gate_H, gate_L, hiRaw_next, stepsSinceEdge_next] = ss_pwm_gate_step( ...
    cnt, dir, ccrUp, ccrDown, hiRaw_prev, stepsSinceEdge_prev, deadTimeFastSteps)
%SS_PWM_GATE_STEP One fast-rate (p.FastTs) step of a single phase's
% high/low-side switch state, matching STM32 timer PWM mode 1 (active
% while counter < compare value, regardless of counting direction) with
% dead-time inserted around every transition.
%
% Call this once per phase (A/B/C) each fast step - each phase has its
% own hiRaw_prev/stepsSinceEdge_prev state, fed back through Unit Delay
% (Z^-1) blocks AT THE FAST RATE, initial condition hiRaw=false,
% stepsSinceEdge=deadTimeFastSteps (so the very first step isn't wrongly
% held in a dead zone).
%
% This is a genuinely stateful, one-fast-step-at-a-time replacement for
% ss_pwm_waveform.m's batch/offline NxN dead-time trick - simpler and
% more natural now that this runs as part of the live simulation instead
% of a one-shot reconstruction: "how many fast steps since the last
% transition" is just a counter, no need to find edges after the fact.
%
% cnt, dir            : ss_pwm_carrier_step.m output, this fast step
% ccrUp, ccrDown       : this phase's compare value for the up-count/
%                        down-count half (ss_calc_duty_and_samplepoints.m's
%                        DmaBuffCCR_up(k)/DmaBuffCCR_down(k), HELD constant
%                        across the whole PWM period via a Rate Transition
%                        block from the slow p.Ts domain)
% hiRaw_prev           : previous fast step's un-gated compare result
%                        (before dead-time), for edge detection
% stepsSinceEdge_prev  : fast steps elapsed since the last transition
% deadTimeFastSteps    : p.DeadTimeFastSteps
%
% gate_H, gate_L       : dead-time-gated high/low-side switch state
% hiRaw_next, stepsSinceEdge_next : feed back to next fast step

if dir > 0
    hiRaw_next = double(cnt < ccrUp);
else
    hiRaw_next = double(cnt < ccrDown);
end

if hiRaw_next ~= hiRaw_prev
    stepsSinceEdge_next = double(0);
else
    stepsSinceEdge_next = double(stepsSinceEdge_prev + 1);
end

inDeadZone = stepsSinceEdge_next < deadTimeFastSteps;

gate_H = double(hiRaw_next & ~inDeadZone);
gate_L = double(~hiRaw_next & ~inDeadZone);

end

== matlab function FOC_core/PWM_Carrier/MATLAB Function4 ==
  data: cnt input; gate_H output double; dir input; ccrUp input; ccrDown input; hiRaw_prev input double; stepsSinceEdge_prev input double; deadTimeFastSteps input; gate_L output double; hiRaw_next output; stepsSinceEdge_next output
function [gate_H, gate_L, hiRaw_next, stepsSinceEdge_next] = ss_pwm_gate_step( ...
    cnt, dir, ccrUp, ccrDown, hiRaw_prev, stepsSinceEdge_prev, deadTimeFastSteps)
%SS_PWM_GATE_STEP One fast-rate (p.FastTs) step of a single phase's
% high/low-side switch state, matching STM32 timer PWM mode 1 (active
% while counter < compare value, regardless of counting direction) with
% dead-time inserted around every transition.
%
% Call this once per phase (A/B/C) each fast step - each phase has its
% own hiRaw_prev/stepsSinceEdge_prev state, fed back through Unit Delay
% (Z^-1) blocks AT THE FAST RATE, initial condition hiRaw=false,
% stepsSinceEdge=deadTimeFastSteps (so the very first step isn't wrongly
% held in a dead zone).
%
% This is a genuinely stateful, one-fast-step-at-a-time replacement for
% ss_pwm_waveform.m's batch/offline NxN dead-time trick - simpler and
% more natural now that this runs as part of the live simulation instead
% of a one-shot reconstruction: "how many fast steps since the last
% transition" is just a counter, no need to find edges after the fact.
%
% cnt, dir            : ss_pwm_carrier_step.m output, this fast step
% ccrUp, ccrDown       : this phase's compare value for the up-count/
%                        down-count half (ss_calc_duty_and_samplepoints.m's
%                        DmaBuffCCR_up(k)/DmaBuffCCR_down(k), HELD constant
%                        across the whole PWM period via a Rate Transition
%                        block from the slow p.Ts domain)
% hiRaw_prev           : previous fast step's un-gated compare result
%                        (before dead-time), for edge detection
% stepsSinceEdge_prev  : fast steps elapsed since the last transition
% deadTimeFastSteps    : p.DeadTimeFastSteps
%
% gate_H, gate_L       : dead-time-gated high/low-side switch state
% hiRaw_next, stepsSinceEdge_next : feed back to next fast step

if dir > 0
    hiRaw_next = double(cnt < ccrUp);
else
    hiRaw_next = double(cnt < ccrDown);
end

if hiRaw_next ~= hiRaw_prev
    stepsSinceEdge_next = double(0);
else
    stepsSinceEdge_next = double(stepsSinceEdge_prev + 1);
end

inDeadZone = stepsSinceEdge_next < deadTimeFastSteps;

gate_H = double(hiRaw_next & ~inDeadZone);
gate_L = double(~hiRaw_next & ~inDeadZone);

end

== matlab function FOC_core/PWM_Carrier/ss_pwm_carrier_step ==
  data: cnt_prev input; cnt_next output; dir_prev input; ticksPerFastStep input; HalfPwmPeriod input; dir_next output
function [cnt_next, dir_next] = ss_pwm_carrier_step(cnt_prev, dir_prev, ticksPerFastStep, HalfPwmPeriod)
%SS_PWM_CARRIER_STEP One fast-rate (p.FastTs) step of the real TIM1
% center-aligned up-down counter, running underneath the whole p.Ts-rate
% model - NOT a firmware port (the real counter is free-running hardware,
% not software), just this simulation's stand-in for it.
%
% Advances the counter by ticksPerFastStep each fast step and reflects
% direction at 0 and HalfPwmPeriod, producing the same triangle-wave
% counter TIM1 actually runs (0 -> HalfPwmPeriod -> 0, repeating every
% p.Ts). Run this in a subsystem at p.FastTs (see ss_params.m's "PWM
% carrier" section) - NOT at the model's main p.Ts rate.
%
% cnt_prev, dir_prev : counter state (ticks, +1/-1) - feed back through
%                       two Unit Delay (Z^-1) blocks AT THE FAST RATE,
%                       initial condition cnt=0, dir=+1
% ticksPerFastStep    : p.TicksPerFastStep
% HalfPwmPeriod       : p.HalfPwmPeriod (ARR, timer ticks)

cnt_raw = cnt_prev + dir_prev * ticksPerFastStep;

if cnt_raw >= HalfPwmPeriod
    cnt_next = HalfPwmPeriod - (cnt_raw - HalfPwmPeriod);
    dir_next = -1;
elseif cnt_raw <= 0
    cnt_next = -cnt_raw;
    dir_next = 1;
else
    cnt_next = cnt_raw;
    dir_next = dir_prev;
end

end

== matlab function FOC_core/compressorLoadProfile/MATLAB Function1 ==
  data: theta_mech_prev input; theta_mech_next output; wmech input; Ts input
function theta_mech_next = ss_mech_angle_step(theta_mech_prev, wmech, Ts)
%SS_MECH_ANGLE_STEP Integrates the rotor/crankshaft's absolute MECHANICAL
% angle (wrapped [0, 2*pi) - one full mechanical revolution). NOT the
% same as ss_theta_step.m's electrical angle, which wraps
% p.MotorPolePairs times faster and loses track of which mechanical
% revolution you're in - needed here because a compressor's load torque
% repeats once per mechanical revolution (crank angle), not once per
% electrical cycle.
%
% theta_mech_prev : previous period's mechanical angle - feed back
%                   through a Unit Delay (Z^-1), initial condition 0
% wmech           : ss_mechanical_model.m's own wmech_next, mechanical
%                   rad/s - UNSCALED (do not multiply by pole_pairs; that
%                   conversion is only for the electrical angle/back-EMF
%                   chain, see ss_theta_step.m / ss_bemf_lookup.m)
% Ts              : p.Ts

theta_mech_next = mod(theta_mech_prev + wmech * Ts, 2*pi);

end
